simulink model "MLI17"  (R2025a)
settings: Solver=ode45  StartTime=0.0  StopTime=.5  RelTol=1e-3  EnableMultiTasking=on
libraries: spsMosfetLib x12, spsSeriesRLCBranchLib x11, spsVoltageMeasurementLib x10, spsDiodeLib x8, spsControlledCurrentSourceLib x8, spsCurrentMeasurementLib x8, spsParallelRLCLoadLib x1, spspowerguiLib x1
(part 2 of 2)

== system MLI17/PV array4/Subsystem1/Subsystem ==
  Isc : Inport
  S : Inport  Port=2
  Tamb : Inport  Port=3
  Tref : Inport  Port=4
  Add : Sum
  Add1 : Sum
  Constant1 : Constant
  Constant2 : Constant  Value=0.03
  Divide : Product  Inputs=*/
  Product{,1..3} (4 alike) : Product  RndMeth=Zero
  Sref : Constant  Value=1000
  Subtract : Sum  Inputs=+-
  a : Constant  Value=0.0025
  Isc' : Outport
  wires:
  Add1/1 -> Subtract/1
  Tamb/1 -> Add1/2
  Product3/1 -> Add1/1
  Constant2/1 -> Product3/2
  Tref/1 -> Subtract/2
  Divide/1 -> Isc'/1
  Sref/1 -> Divide/2
  Product2/1 -> Divide/1
  Add/1 -> Product2/2
  Product1/1 -> Product2/1
  S/1 -> Product3/1, Product1/2
  Isc/1 -> Product1/1
  Product/1 -> Add/1
  Constant1/1 -> Add/2
  a/1 -> Product/1
  Subtract/1 -> Product/2

== system MLI17/PV array4/Subsystem1/Subsystem1 ==
  S : Inport
  Tamb : Inport  Port=2
  Tref : Inport  Port=3
  Voc : Inport  Port=4
  Add : Sum
  Add1 : Sum
  Constant1 : Constant
  Constant2 : Constant
  Constant3 : Constant
  Constant4 : Constant  Value=0.03
  Constant5 : Constant  Value=0.2
  Divide : Product  Inputs=*/
  Product{,1..4} (5 alike) : Product  RndMeth=Zero
  Sref : Constant  Value=1000
  Subtract : Sum  Inputs=+-
  Subtract1 : Sum  Inputs=+-
  Subtract2 : Sum  Inputs=+-
  c : Constant  Value=0.00288
  Voc' : Outport
  wires:
  Constant5/1 -> Product1/1
  Add1/1 -> Subtract/1
  Tamb/1 -> Add1/2
  Product4/1 -> Add1/1
  Constant4/1 -> Product4/2
  Constant3/1 -> Subtract2/2
  Divide/1 -> Subtract2/1
  Sref/1 -> Divide/2
  S/1 -> Product4/1, Divide/1
  Product3/1 -> Voc'/1
  Voc/1 -> Product3/2
  Product2/1 -> Product3/1
  Add/1 -> Product2/1
  Subtract1/1 -> Product2/2
  Product1/1 -> Add/2
  Constant2/1 -> Add/1
  Subtract2/1 -> Product1/2
  Product/1 -> Subtract1/2
  Constant1/1 -> Subtract1/1
  Subtract/1 -> Product/2
  c/1 -> Product/1
  Tref/1 -> Subtract/2

== system MLI17/PV array4/Subsystem1/Subsystem2 ==
  Im : Inport
  S : Inport  Port=2
  Tamb : Inport  Port=3
  Tref : Inport  Port=4
  Add : Sum
  Add1 : Sum
  Constant1 : Constant
  Constant2 : Constant  Value=0.03
  Divide : Product  Inputs=*/
  Product{,1..3} (4 alike) : Product  RndMeth=Zero
  Sref : Constant  Value=1000
  Subtract : Sum  Inputs=+-
  a : Constant  Value=0.0025
  Im' : Outport
  wires:
  Add1/1 -> Subtract/1
  Tamb/1 -> Add1/2
  Product3/1 -> Add1/1
  Constant2/1 -> Product3/2
  Tref/1 -> Subtract/2
  Divide/1 -> Im'/1
  Sref/1 -> Divide/2
  Product2/1 -> Divide/1
  Add/1 -> Product2/2
  Product1/1 -> Product2/1
  S/1 -> Product3/1, Product1/2
  Im/1 -> Product1/1
  Product/1 -> Add/1
  Constant1/1 -> Add/2
  a/1 -> Product/1
  Subtract/1 -> Product/2

== system MLI17/PV array4/Subsystem1/Subsystem3 ==
  S : Inport
  Tamb : Inport  Port=2
  Tref : Inport  Port=3
  Vm : Inport  Port=4
  Add : Sum
  Add1 : Sum
  Constant1 : Constant
  Constant2 : Constant
  Constant3 : Constant
  Constant4 : Constant  Value=0.03
  Constant5 : Constant  Value=0.2
  Divide : Product  Inputs=*/
  Product{,1..4} (5 alike) : Product  RndMeth=Zero
  Sref : Constant  Value=1000
  Subtract : Sum  Inputs=+-
  Subtract1 : Sum  Inputs=+-
  Subtract2 : Sum  Inputs=+-
  c : Constant  Value=0.00288
  Vm' : Outport
  wires:
  Constant5/1 -> Product1/1
  Add1/1 -> Subtract/1
  Tamb/1 -> Add1/2
  Product4/1 -> Add1/1
  Constant4/1 -> Product4/2
  Constant3/1 -> Subtract2/2
  Divide/1 -> Subtract2/1
  Sref/1 -> Divide/2
  S/1 -> Product4/1, Divide/1
  Product3/1 -> Vm'/1
  Vm/1 -> Product3/2
  Product2/1 -> Product3/1
  Add/1 -> Product2/1
  Subtract1/1 -> Product2/2
  Product1/1 -> Add/2
  Constant2/1 -> Add/1
  Subtract2/1 -> Product1/2
  Product/1 -> Subtract1/2
  Constant1/1 -> Subtract1/1
  Subtract/1 -> Product/2
  c/1 -> Product/1
  Tref/1 -> Subtract/2

== system MLI17/PV array4/Subsystem1/Subsystem5 ==
  C2 : Inport
  Vm : Inport  Port=2
  Voc : Inport  Port=3
  Im : Inport  Port=4
  Isc : Inport  Port=5
  Constant : Constant
  Constant1 : Constant  Value=-1
  Divide : Product  Inputs=*/
  Divide1 : Product  Inputs=*/
  Math Function : Math  SignedPower=on
  Product : Product  RndMeth=Zero
  Product1 : Product  RndMeth=Zero
  Product2 : Product  RndMeth=Zero
  Subtract : Sum  Inputs=+-
  C1 : Outport
  wires:
  Divide/1 -> Subtract/2
  Constant/1 -> Subtract/1
  Isc/1 -> Divide/2
  Im/1 -> Divide/1
  C2/1 -> Product/1
  Voc/1 -> Product/2
  Vm/1 -> Divide1/1
  Product2/1 -> C1/1
  Subtract/1 -> Product2/2
  Math Function/1 -> Product2/1
  Product1/1 -> Math Function/1
  Constant1/1 -> Product1/1
  Divide1/1 -> Product1/2
  Product/1 -> Divide1/2

== system MLI17/PV array4/Subsystem1/Subsystem6 ==
  Im : Inport
  Isc : Inport  Port=2
  Vm : Inport  Port=3
  Voc : Inport  Port=4
  Constant : Constant
  Constant1 : Constant
  Divide : Product  Inputs=*/
  Divide1 : Product  Inputs=*/
  Divide2 : Product  Inputs=*/
  Math Function : Math  Operator=log  SignedPower=on
  Subtract : Sum  Inputs=+-
  Subtract1 : Sum  Inputs=+-
  C2 : Outport
  wires:
  Math Function/1 -> Divide2/2
  Subtract/1 -> Divide2/1
  Subtract1/1 -> Math Function/1
  Isc/1 -> Divide1/2
  Im/1 -> Divide1/1
  Voc/1 -> Divide/2
  Vm/1 -> Divide/1
  Divide2/1 -> C2/1
  Divide1/1 -> Subtract1/2
  Constant1/1 -> Subtract1/1
  Constant/1 -> Subtract/2
  Divide/1 -> Subtract/1

== system MLI17/PV array5/Subsystem1/Subsystem ==
  Isc : Inport
  S : Inport  Port=2
  Tamb : Inport  Port=3
  Tref : Inport  Port=4
  Add : Sum
  Add1 : Sum
  Constant1 : Constant
  Constant2 : Constant  Value=0.03
  Divide : Product  Inputs=*/
  Product{,1..3} (4 alike) : Product  RndMeth=Zero
  Sref : Constant  Value=1000
  Subtract : Sum  Inputs=+-
  a : Constant  Value=0.0025
  Isc' : Outport
  wires:
  Subtract/1 -> Product/2
  a/1 -> Product/1
  Constant1/1 -> Add/2
  Product/1 -> Add/1
  Isc/1 -> Product1/1
  S/1 -> Product1/2, Product3/1
  Product1/1 -> Product2/1
  Add/1 -> Product2/2
  Product2/1 -> Divide/1
  Sref/1 -> Divide/2
  Divide/1 -> Isc'/1
  Tref/1 -> Subtract/2
  Constant2/1 -> Product3/2
  Product3/1 -> Add1/1
  Tamb/1 -> Add1/2
  Add1/1 -> Subtract/1

== system MLI17/PV array5/Subsystem1/Subsystem1 ==
  S : Inport
  Tamb : Inport  Port=2
  Tref : Inport  Port=3
  Voc : Inport  Port=4
  Add : Sum
  Add1 : Sum
  Constant1 : Constant
  Constant2 : Constant
  Constant3 : Constant
  Constant4 : Constant  Value=0.03
  Constant5 : Constant  Value=0.2
  Divide : Product  Inputs=*/
  Product{,1..4} (5 alike) : Product  RndMeth=Zero
  Sref : Constant  Value=1000
  Subtract : Sum  Inputs=+-
  Subtract1 : Sum  Inputs=+-
  Subtract2 : Sum  Inputs=+-
  c : Constant  Value=0.00288
  Voc' : Outport
  wires:
  Tref/1 -> Subtract/2
  c/1 -> Product/1
  Subtract/1 -> Product/2
  Constant1/1 -> Subtract1/1
  Product/1 -> Subtract1/2
  Subtract2/1 -> Product1/2
  Constant2/1 -> Add/1
  Product1/1 -> Add/2
  Subtract1/1 -> Product2/2
  Add/1 -> Product2/1
  Product2/1 -> Product3/1
  Voc/1 -> Product3/2
  Product3/1 -> Voc'/1
  S/1 -> Divide/1, Product4/1
  Sref/1 -> Divide/2
  Divide/1 -> Subtract2/1
  Constant3/1 -> Subtract2/2
  Constant4/1 -> Product4/2
  Product4/1 -> Add1/1
  Tamb/1 -> Add1/2
  Add1/1 -> Subtract/1
  Constant5/1 -> Product1/1

== system MLI17/PV array5/Subsystem1/Subsystem2 ==
  Im : Inport
  S : Inport  Port=2
  Tamb : Inport  Port=3
  Tref : Inport  Port=4
  Add : Sum
  Add1 : Sum
  Constant1 : Constant
  Constant2 : Constant  Value=0.03
  Divide : Product  Inputs=*/
  Product{,1..3} (4 alike) : Product  RndMeth=Zero
  Sref : Constant  Value=1000
  Subtract : Sum  Inputs=+-
  a : Constant  Value=0.0025
  Im' : Outport
  wires:
  Subtract/1 -> Product/2
  a/1 -> Product/1
  Constant1/1 -> Add/2
  Product/1 -> Add/1
  Im/1 -> Product1/1
  S/1 -> Product1/2, Product3/1
  Product1/1 -> Product2/1
  Add/1 -> Product2/2
  Product2/1 -> Divide/1
  Sref/1 -> Divide/2
  Divide/1 -> Im'/1
  Tref/1 -> Subtract/2
  Constant2/1 -> Product3/2
  Product3/1 -> Add1/1
  Tamb/1 -> Add1/2
  Add1/1 -> Subtract/1

== system MLI17/PV array5/Subsystem1/Subsystem3 ==
  S : Inport
  Tamb : Inport  Port=2
  Tref : Inport  Port=3
  Vm : Inport  Port=4
  Add : Sum
  Add1 : Sum
  Constant1 : Constant
  Constant2 : Constant
  Constant3 : Constant
  Constant4 : Constant  Value=0.03
  Constant5 : Constant  Value=0.2
  Divide : Product  Inputs=*/
  Product{,1..4} (5 alike) : Product  RndMeth=Zero
  Sref : Constant  Value=1000
  Subtract : Sum  Inputs=+-
  Subtract1 : Sum  Inputs=+-
  Subtract2 : Sum  Inputs=+-
  c : Constant  Value=0.00288
  Vm' : Outport
  wires:
  Tref/1 -> Subtract/2
  c/1 -> Product/1
  Subtract/1 -> Product/2
  Constant1/1 -> Subtract1/1
  Product/1 -> Subtract1/2
  Subtract2/1 -> Product1/2
  Constant2/1 -> Add/1
  Product1/1 -> Add/2
  Subtract1/1 -> Product2/2
  Add/1 -> Product2/1
  Product2/1 -> Product3/1
  Vm/1 -> Product3/2
  Product3/1 -> Vm'/1
  S/1 -> Divide/1, Product4/1
  Sref/1 -> Divide/2
  Divide/1 -> Subtract2/1
  Constant3/1 -> Subtract2/2
  Constant4/1 -> Product4/2
  Product4/1 -> Add1/1
  Tamb/1 -> Add1/2
  Add1/1 -> Subtract/1
  Constant5/1 -> Product1/1

== system MLI17/PV array5/Subsystem1/Subsystem5 ==
  C2 : Inport
  Vm : Inport  Port=2
  Voc : Inport  Port=3
  Im : Inport  Port=4
  Isc : Inport  Port=5
  Constant : Constant
  Constant1 : Constant  Value=-1
  Divide : Product  Inputs=*/
  Divide1 : Product  Inputs=*/
  Math Function : Math  SignedPower=on
  Product : Product  RndMeth=Zero
  Product1 : Product  RndMeth=Zero
  Product2 : Product  RndMeth=Zero
  Subtract : Sum  Inputs=+-
  C1 : Outport
  wires:
  Product/1 -> Divide1/2
  Divide1/1 -> Product1/2
  Constant1/1 -> Product1/1
  Product1/1 -> Math Function/1
  Math Function/1 -> Product2/1
  Subtract/1 -> Product2/2
  Product2/1 -> C1/1
  Vm/1 -> Divide1/1
  Voc/1 -> Product/2
  C2/1 -> Product/1
  Im/1 -> Divide/1
  Isc/1 -> Divide/2
  Constant/1 -> Subtract/1
  Divide/1 -> Subtract/2

== system MLI17/PV array5/Subsystem1/Subsystem6 ==
  Im : Inport
  Isc : Inport  Port=2
  Vm : Inport  Port=3
  Voc : Inport  Port=4
  Constant : Constant
  Constant1 : Constant
  Divide : Product  Inputs=*/
  Divide1 : Product  Inputs=*/
  Divide2 : Product  Inputs=*/
  Math Function : Math  Operator=log  SignedPower=on
  Subtract : Sum  Inputs=+-
  Subtract1 : Sum  Inputs=+-
  C2 : Outport
  wires:
  Divide/1 -> Subtract/1
  Constant/1 -> Subtract/2
  Constant1/1 -> Subtract1/1
  Divide1/1 -> Subtract1/2
  Divide2/1 -> C2/1
  Vm/1 -> Divide/1
  Voc/1 -> Divide/2
  Im/1 -> Divide1/1
  Isc/1 -> Divide1/2
  Subtract1/1 -> Math Function/1
  Subtract/1 -> Divide2/1
  Math Function/1 -> Divide2/2

== system MLI17/PV array6/Subsystem1/Subsystem ==
  Isc : Inport
  S : Inport  Port=2
  Tamb : Inport  Port=3
  Tref : Inport  Port=4
  Add : Sum
  Add1 : Sum
  Constant1 : Constant
  Constant2 : Constant  Value=0.03
  Divide : Product  Inputs=*/
  Product{,1..3} (4 alike) : Product  RndMeth=Zero
  Sref : Constant  Value=1000
  Subtract : Sum  Inputs=+-
  a : Constant  Value=0.0025
  Isc' : Outport
  wires:
  Add1/1 -> Subtract/1
  Tamb/1 -> Add1/2
  Product3/1 -> Add1/1
  Constant2/1 -> Product3/2
  Tref/1 -> Subtract/2
  Divide/1 -> Isc'/1
  Sref/1 -> Divide/2
  Product2/1 -> Divide/1
  Add/1 -> Product2/2
  Product1/1 -> Product2/1
  S/1 -> Product3/1, Product1/2
  Isc/1 -> Product1/1
  Product/1 -> Add/1
  Constant1/1 -> Add/2
  a/1 -> Product/1
  Subtract/1 -> Product/2

== system MLI17/PV array6/Subsystem1/Subsystem1 ==
  S : Inport
  Tamb : Inport  Port=2
  Tref : Inport  Port=3
  Voc : Inport  Port=4
  Add : Sum
  Add1 : Sum
  Constant1 : Constant
  Constant2 : Constant
  Constant3 : Constant
  Constant4 : Constant  Value=0.03
  Constant5 : Constant  Value=0.2
  Divide : Product  Inputs=*/
  Product{,1..4} (5 alike) : Product  RndMeth=Zero
  Sref : Constant  Value=1000
  Subtract : Sum  Inputs=+-
  Subtract1 : Sum  Inputs=+-
  Subtract2 : Sum  Inputs=+-
  c : Constant  Value=0.00288
  Voc' : Outport
  wires:
  Constant5/1 -> Product1/1
  Add1/1 -> Subtract/1
  Tamb/1 -> Add1/2
  Product4/1 -> Add1/1
  Constant4/1 -> Product4/2
  Constant3/1 -> Subtract2/2
  Divide/1 -> Subtract2/1
  Sref/1 -> Divide/2
  S/1 -> Product4/1, Divide/1
  Product3/1 -> Voc'/1
  Voc/1 -> Product3/2
  Product2/1 -> Product3/1
  Add/1 -> Product2/1
  Subtract1/1 -> Product2/2
  Product1/1 -> Add/2
  Constant2/1 -> Add/1
  Subtract2/1 -> Product1/2
  Product/1 -> Subtract1/2
  Constant1/1 -> Subtract1/1
  Subtract/1 -> Product/2
  c/1 -> Product/1
  Tref/1 -> Subtract/2

== system MLI17/PV array6/Subsystem1/Subsystem2 ==
  Im : Inport
  S : Inport  Port=2
  Tamb : Inport  Port=3
  Tref : Inport  Port=4
  Add : Sum
  Add1 : Sum
  Constant1 : Constant
  Constant2 : Constant  Value=0.03
  Divide : Product  Inputs=*/
  Product{,1..3} (4 alike) : Product  RndMeth=Zero
  Sref : Constant  Value=1000
  Subtract : Sum  Inputs=+-
  a : Constant  Value=0.0025
  Im' : Outport
  wires:
  Add1/1 -> Subtract/1
  Tamb/1 -> Add1/2
  Product3/1 -> Add1/1
  Constant2/1 -> Product3/2
  Tref/1 -> Subtract/2
  Divide/1 -> Im'/1
  Sref/1 -> Divide/2
  Product2/1 -> Divide/1
  Add/1 -> Product2/2
  Product1/1 -> Product2/1
  S/1 -> Product3/1, Product1/2
  Im/1 -> Product1/1
  Product/1 -> Add/1
  Constant1/1 -> Add/2
  a/1 -> Product/1
  Subtract/1 -> Product/2

== system MLI17/PV array6/Subsystem1/Subsystem3 ==
  S : Inport
  Tamb : Inport  Port=2
  Tref : Inport  Port=3
  Vm : Inport  Port=4
  Add : Sum
  Add1 : Sum
  Constant1 : Constant
  Constant2 : Constant
  Constant3 : Constant
  Constant4 : Constant  Value=0.03
  Constant5 : Constant  Value=0.2
  Divide : Product  Inputs=*/
  Product{,1..4} (5 alike) : Product  RndMeth=Zero
  Sref : Constant  Value=1000
  Subtract : Sum  Inputs=+-
  Subtract1 : Sum  Inputs=+-
  Subtract2 : Sum  Inputs=+-
  c : Constant  Value=0.00288
  Vm' : Outport
  wires:
  Constant5/1 -> Product1/1
  Add1/1 -> Subtract/1
  Tamb/1 -> Add1/2
  Product4/1 -> Add1/1
  Constant4/1 -> Product4/2
  Constant3/1 -> Subtract2/2
  Divide/1 -> Subtract2/1
  Sref/1 -> Divide/2
  S/1 -> Product4/1, Divide/1
  Product3/1 -> Vm'/1
  Vm/1 -> Product3/2
  Product2/1 -> Product3/1
  Add/1 -> Product2/1
  Subtract1/1 -> Product2/2
  Product1/1 -> Add/2
  Constant2/1 -> Add/1
  Subtract2/1 -> Product1/2
  Product/1 -> Subtract1/2
  Constant1/1 -> Subtract1/1
  Subtract/1 -> Product/2
  c/1 -> Product/1
  Tref/1 -> Subtract/2

== system MLI17/PV array6/Subsystem1/Subsystem5 ==
  C2 : Inport
  Vm : Inport  Port=2
  Voc : Inport  Port=3
  Im : Inport  Port=4
  Isc : Inport  Port=5
  Constant : Constant
  Constant1 : Constant  Value=-1
  Divide : Product  Inputs=*/
  Divide1 : Product  Inputs=*/
  Math Function : Math  SignedPower=on
  Product : Product  RndMeth=Zero
  Product1 : Product  RndMeth=Zero
  Product2 : Product  RndMeth=Zero
  Subtract : Sum  Inputs=+-
  C1 : Outport
  wires:
  Divide/1 -> Subtract/2
  Constant/1 -> Subtract/1
  Isc/1 -> Divide/2
  Im/1 -> Divide/1
  C2/1 -> Product/1
  Voc/1 -> Product/2
  Vm/1 -> Divide1/1
  Product2/1 -> C1/1
  Subtract/1 -> Product2/2
  Math Function/1 -> Product2/1
  Product1/1 -> Math Function/1
  Constant1/1 -> Product1/1
  Divide1/1 -> Product1/2
  Product/1 -> Divide1/2

== system MLI17/PV array6/Subsystem1/Subsystem6 ==
  Im : Inport
  Isc : Inport  Port=2
  Vm : Inport  Port=3
  Voc : Inport  Port=4
  Constant : Constant
  Constant1 : Constant
  Divide : Product  Inputs=*/
  Divide1 : Product  Inputs=*/
  Divide2 : Product  Inputs=*/
  Math Function : Math  Operator=log  SignedPower=on
  Subtract : Sum  Inputs=+-
  Subtract1 : Sum  Inputs=+-
  C2 : Outport
  wires:
  Math Function/1 -> Divide2/2
  Subtract/1 -> Divide2/1
  Subtract1/1 -> Math Function/1
  Isc/1 -> Divide1/2
  Im/1 -> Divide1/1
  Voc/1 -> Divide/2
  Vm/1 -> Divide/1
  Divide2/1 -> C2/1
  Divide1/1 -> Subtract1/2
  Constant1/1 -> Subtract1/1
  Constant/1 -> Subtract/2
  Divide/1 -> Subtract/1

== system MLI17/PV array7/Subsystem1/Subsystem ==
  Isc : Inport
  S : Inport  Port=2
  Tamb : Inport  Port=3
  Tref : Inport  Port=4
  Add : Sum
  Add1 : Sum
  Constant1 : Constant
  Constant2 : Constant  Value=0.03
  Divide : Product  Inputs=*/
  Product{,1..3} (4 alike) : Product  RndMeth=Zero
  Sref : Constant  Value=1000
  Subtract : Sum  Inputs=+-
  a : Constant  Value=0.0025
  Isc' : Outport
  wires:
  Subtract/1 -> Product/2
  a/1 -> Product/1
  Constant1/1 -> Add/2
  Product/1 -> Add/1
  Isc/1 -> Product1/1
  S/1 -> Product1/2, Product3/1
  Product1/1 -> Product2/1
  Add/1 -> Product2/2
  Product2/1 -> Divide/1
  Sref/1 -> Divide/2
  Divide/1 -> Isc'/1
  Tref/1 -> Subtract/2
  Constant2/1 -> Product3/2
  Product3/1 -> Add1/1
  Tamb/1 -> Add1/2
  Add1/1 -> Subtract/1

== system MLI17/PV array7/Subsystem1/Subsystem1 ==
  S : Inport
  Tamb : Inport  Port=2
  Tref : Inport  Port=3
  Voc : Inport  Port=4
  Add : Sum
  Add1 : Sum
  Constant1 : Constant
  Constant2 : Constant
  Constant3 : Constant
  Constant4 : Constant  Value=0.03
  Constant5 : Constant  Value=0.2
  Divide : Product  Inputs=*/
  Product{,1..4} (5 alike) : Product  RndMeth=Zero
  Sref : Constant  Value=1000
  Subtract : Sum  Inputs=+-
  Subtract1 : Sum  Inputs=+-
  Subtract2 : Sum  Inputs=+-
  c : Constant  Value=0.00288
  Voc' : Outport
  wires:
  Tref/1 -> Subtract/2
  c/1 -> Product/1
  Subtract/1 -> Product/2
  Constant1/1 -> Subtract1/1
  Product/1 -> Subtract1/2
  Subtract2/1 -> Product1/2
  Constant2/1 -> Add/1
  Product1/1 -> Add/2
  Subtract1/1 -> Product2/2
  Add/1 -> Product2/1
  Product2/1 -> Product3/1
  Voc/1 -> Product3/2
  Product3/1 -> Voc'/1
  S/1 -> Divide/1, Product4/1
  Sref/1 -> Divide/2
  Divide/1 -> Subtract2/1
  Constant3/1 -> Subtract2/2
  Constant4/1 -> Product4/2
  Product4/1 -> Add1/1
  Tamb/1 -> Add1/2
  Add1/1 -> Subtract/1
  Constant5/1 -> Product1/1

== system MLI17/PV array7/Subsystem1/Subsystem2 ==
  Im : Inport
  S : Inport  Port=2
  Tamb : Inport  Port=3
  Tref : Inport  Port=4
  Add : Sum
  Add1 : Sum
  Constant1 : Constant
  Constant2 : Constant  Value=0.03
  Divide : Product  Inputs=*/
  Product{,1..3} (4 alike) : Product  RndMeth=Zero
  Sref : Constant  Value=1000
  Subtract : Sum  Inputs=+-
  a : Constant  Value=0.0025
  Im' : Outport
  wires:
  Subtract/1 -> Product/2
  a/1 -> Product/1
  Constant1/1 -> Add/2
  Product/1 -> Add/1
  Im/1 -> Product1/1
  S/1 -> Product1/2, Product3/1
  Product1/1 -> Product2/1
  Add/1 -> Product2/2
  Product2/1 -> Divide/1
  Sref/1 -> Divide/2
  Divide/1 -> Im'/1
  Tref/1 -> Subtract/2
  Constant2/1 -> Product3/2
  Product3/1 -> Add1/1
  Tamb/1 -> Add1/2
  Add1/1 -> Subtract/1

== system MLI17/PV array7/Subsystem1/Subsystem3 ==
  S : Inport
  Tamb : Inport  Port=2
  Tref : Inport  Port=3
  Vm : Inport  Port=4
  Add : Sum
  Add1 : Sum
  Constant1 : Constant
  Constant2 : Constant
  Constant3 : Constant
  Constant4 : Constant  Value=0.03
  Constant5 : Constant  Value=0.2
  Divide : Product  Inputs=*/
  Product{,1..4} (5 alike) : Product  RndMeth=Zero
  Sref : Constant  Value=1000
  Subtract : Sum  Inputs=+-
  Subtract1 : Sum  Inputs=+-
  Subtract2 : Sum  Inputs=+-
  c : Constant  Value=0.00288
  Vm' : Outport
  wires:
  Tref/1 -> Subtract/2
  c/1 -> Product/1
  Subtract/1 -> Product/2
  Constant1/1 -> Subtract1/1
  Product/1 -> Subtract1/2
  Subtract2/1 -> Product1/2
  Constant2/1 -> Add/1
  Product1/1 -> Add/2
  Subtract1/1 -> Product2/2
  Add/1 -> Product2/1
  Product2/1 -> Product3/1
  Vm/1 -> Product3/2
  Product3/1 -> Vm'/1
  S/1 -> Divide/1, Product4/1
  Sref/1 -> Divide/2
  Divide/1 -> Subtract2/1
  Constant3/1 -> Subtract2/2
  Constant4/1 -> Product4/2
  Product4/1 -> Add1/1
  Tamb/1 -> Add1/2
  Add1/1 -> Subtract/1
  Constant5/1 -> Product1/1

== system MLI17/PV array7/Subsystem1/Subsystem5 ==
  C2 : Inport
  Vm : Inport  Port=2
  Voc : Inport  Port=3
  Im : Inport  Port=4
  Isc : Inport  Port=5
  Constant : Constant
  Constant1 : Constant  Value=-1
  Divide : Product  Inputs=*/
  Divide1 : Product  Inputs=*/
  Math Function : Math  SignedPower=on
  Product : Product  RndMeth=Zero
  Product1 : Product  RndMeth=Zero
  Product2 : Product  RndMeth=Zero
  Subtract : Sum  Inputs=+-
  C1 : Outport
  wires:
  Product/1 -> Divide1/2
  Divide1/1 -> Product1/2
  Constant1/1 -> Product1/1
  Product1/1 -> Math Function/1
  Math Function/1 -> Product2/1
  Subtract/1 -> Product2/2
  Product2/1 -> C1/1
  Vm/1 -> Divide1/1
  Voc/1 -> Product/2
  C2/1 -> Product/1
  Im/1 -> Divide/1
  Isc/1 -> Divide/2
  Constant/1 -> Subtract/1
  Divide/1 -> Subtract/2

== system MLI17/PV array7/Subsystem1/Subsystem6 ==
  Im : Inport
  Isc : Inport  Port=2
  Vm : Inport  Port=3
  Voc : Inport  Port=4
  Constant : Constant
  Constant1 : Constant
  Divide : Product  Inputs=*/
  Divide1 : Product  Inputs=*/
  Divide2 : Product  Inputs=*/
  Math Function : Math  Operator=log  SignedPower=on
  Subtract : Sum  Inputs=+-
  Subtract1 : Sum  Inputs=+-
  C2 : Outport
  wires:
  Divide/1 -> Subtract/1
  Constant/1 -> Subtract/2
  Constant1/1 -> Subtract1/1
  Divide1/1 -> Subtract1/2
  Divide2/1 -> C2/1
  Vm/1 -> Divide/1
  Voc/1 -> Divide/2
  Im/1 -> Divide1/1
  Isc/1 -> Divide1/2
  Subtract1/1 -> Math Function/1
  Subtract/1 -> Divide2/1
  Math Function/1 -> Divide2/2

== system MLI17/PV array8/Subsystem1/Subsystem ==
  Isc : Inport
  S : Inport  Port=2
  Tamb : Inport  Port=3
  Tref : Inport  Port=4
  Add : Sum
  Add1 : Sum
  Constant1 : Constant
  Constant2 : Constant  Value=0.03
  Divide : Product  Inputs=*/
  Product{,1..3} (4 alike) : Product  RndMeth=Zero
  Sref : Constant  Value=1000
  Subtract : Sum  Inputs=+-
  a : Constant  Value=0.0025
  Isc' : Outport
  wires:
  Add1/1 -> Subtract/1
  Tamb/1 -> Add1/2
  Product3/1 -> Add1/1
  Constant2/1 -> Product3/2
  Tref/1 -> Subtract/2
  Divide/1 -> Isc'/1
  Sref/1 -> Divide/2
  Product2/1 -> Divide/1
  Add/1 -> Product2/2
  Product1/1 -> Product2/1
  S/1 -> Product3/1, Product1/2
  Isc/1 -> Product1/1
  Product/1 -> Add/1
  Constant1/1 -> Add/2
  a/1 -> Product/1
  Subtract/1 -> Product/2

== system MLI17/PV array8/Subsystem1/Subsystem1 ==
  S : Inport
  Tamb : Inport  Port=2
  Tref : Inport  Port=3
  Voc : Inport  Port=4
  Add : Sum
  Add1 : Sum
  Constant1 : Constant
  Constant2 : Constant
  Constant3 : Constant
  Constant4 : Constant  Value=0.03
  Constant5 : Constant  Value=0.2
  Divide : Product  Inputs=*/
  Product{,1..4} (5 alike) : Product  RndMeth=Zero
  Sref : Constant  Value=1000
  Subtract : Sum  Inputs=+-
  Subtract1 : Sum  Inputs=+-
  Subtract2 : Sum  Inputs=+-
  c : Constant  Value=0.00288
  Voc' : Outport
  wires:
  Constant5/1 -> Product1/1
  Add1/1 -> Subtract/1
  Tamb/1 -> Add1/2
  Product4/1 -> Add1/1
  Constant4/1 -> Product4/2
  Constant3/1 -> Subtract2/2
  Divide/1 -> Subtract2/1
  Sref/1 -> Divide/2
  S/1 -> Product4/1, Divide/1
  Product3/1 -> Voc'/1
  Voc/1 -> Product3/2
  Product2/1 -> Product3/1
  Add/1 -> Product2/1
  Subtract1/1 -> Product2/2
  Product1/1 -> Add/2
  Constant2/1 -> Add/1
  Subtract2/1 -> Product1/2
  Product/1 -> Subtract1/2
  Constant1/1 -> Subtract1/1
  Subtract/1 -> Product/2
  c/1 -> Product/1
  Tref/1 -> Subtract/2

== system MLI17/PV array8/Subsystem1/Subsystem2 ==
  Im : Inport
  S : Inport  Port=2
  Tamb : Inport  Port=3
  Tref : Inport  Port=4
  Add : Sum
  Add1 : Sum
  Constant1 : Constant
  Constant2 : Constant  Value=0.03
  Divide : Product  Inputs=*/
  Product{,1..3} (4 alike) : Product  RndMeth=Zero
  Sref : Constant  Value=1000
  Subtract : Sum  Inputs=+-
  a : Constant  Value=0.0025
  Im' : Outport
  wires:
  Add1/1 -> Subtract/1
  Tamb/1 -> Add1/2
  Product3/1 -> Add1/1
  Constant2/1 -> Product3/2
  Tref/1 -> Subtract/2
  Divide/1 -> Im'/1
  Sref/1 -> Divide/2
  Product2/1 -> Divide/1
  Add/1 -> Product2/2
  Product1/1 -> Product2/1
  S/1 -> Product3/1, Product1/2
  Im/1 -> Product1/1
  Product/1 -> Add/1
  Constant1/1 -> Add/2
  a/1 -> Product/1
  Subtract/1 -> Product/2

== system MLI17/PV array8/Subsystem1/Subsystem3 ==
  S : Inport
  Tamb : Inport  Port=2
  Tref : Inport  Port=3
  Vm : Inport  Port=4
  Add : Sum
  Add1 : Sum
  Constant1 : Constant
  Constant2 : Constant
  Constant3 : Constant
  Constant4 : Constant  Value=0.03
  Constant5 : Constant  Value=0.2
  Divide : Product  Inputs=*/
  Product{,1..4} (5 alike) : Product  RndMeth=Zero
  Sref : Constant  Value=1000
  Subtract : Sum  Inputs=+-
  Subtract1 : Sum  Inputs=+-
  Subtract2 : Sum  Inputs=+-
  c : Constant  Value=0.00288
  Vm' : Outport
  wires:
  Constant5/1 -> Product1/1
  Add1/1 -> Subtract/1
  Tamb/1 -> Add1/2
  Product4/1 -> Add1/1
  Constant4/1 -> Product4/2
  Constant3/1 -> Subtract2/2
  Divide/1 -> Subtract2/1
  Sref/1 -> Divide/2
  S/1 -> Product4/1, Divide/1
  Product3/1 -> Vm'/1
  Vm/1 -> Product3/2
  Product2/1 -> Product3/1
  Add/1 -> Product2/1
  Subtract1/1 -> Product2/2
  Product1/1 -> Add/2
  Constant2/1 -> Add/1
  Subtract2/1 -> Product1/2
  Product/1 -> Subtract1/2
  Constant1/1 -> Subtract1/1
  Subtract/1 -> Product/2
  c/1 -> Product/1
  Tref/1 -> Subtract/2

== system MLI17/PV array8/Subsystem1/Subsystem5 ==
  C2 : Inport
  Vm : Inport  Port=2
  Voc : Inport  Port=3
  Im : Inport  Port=4
  Isc : Inport  Port=5
  Constant : Constant
  Constant1 : Constant  Value=-1
  Divide : Product  Inputs=*/
  Divide1 : Product  Inputs=*/
  Math Function : Math  SignedPower=on
  Product : Product  RndMeth=Zero
  Product1 : Product  RndMeth=Zero
  Product2 : Product  RndMeth=Zero
  Subtract : Sum  Inputs=+-
  C1 : Outport
  wires:
  Divide/1 -> Subtract/2
  Constant/1 -> Subtract/1
  Isc/1 -> Divide/2
  Im/1 -> Divide/1
  C2/1 -> Product/1
  Voc/1 -> Product/2
  Vm/1 -> Divide1/1
  Product2/1 -> C1/1
  Subtract/1 -> Product2/2
  Math Function/1 -> Product2/1
  Product1/1 -> Math Function/1
  Constant1/1 -> Product1/1
  Divide1/1 -> Product1/2
  Product/1 -> Divide1/2

== system MLI17/PV array8/Subsystem1/Subsystem6 ==
  Im : Inport
  Isc : Inport  Port=2
  Vm : Inport  Port=3
  Voc : Inport  Port=4
  Constant : Constant
  Constant1 : Constant
  Divide : Product  Inputs=*/
  Divide1 : Product  Inputs=*/
  Divide2 : Product  Inputs=*/
  Math Function : Math  Operator=log  SignedPower=on
  Subtract : Sum  Inputs=+-
  Subtract1 : Sum  Inputs=+-
  C2 : Outport
  wires:
  Math Function/1 -> Divide2/2
  Subtract/1 -> Divide2/1
  Subtract1/1 -> Math Function/1
  Isc/1 -> Divide1/2
  Im/1 -> Divide1/1
  Voc/1 -> Divide/2
  Vm/1 -> Divide/1
  Divide2/1 -> C2/1
  Divide1/1 -> Subtract1/2
  Constant1/1 -> Subtract1/1
  Constant/1 -> Subtract/2
  Divide/1 -> Subtract/1
